simulink model "wscc9_transient_stability"  (R2024b)
settings: Solver=VariableStepAuto  StartTime=0.0  StopTime=2  MaxStep=1e-4  RelTol=1e-3
values from neighbouring files (symbols this model uses):
  E1 = E(1)    [wscc9_transient_init.m]
  E2 = E(2)    [wscc9_transient_init.m]
  E3 = E(3)    [wscc9_transient_init.m]
  f = 60    [wscc9_transient_init.m]
  H = [23.645 ; 6.4 ; 3.01]    [wscc9_transient_init.m]
  Pm1 = (Pg(1,1))    [wscc9_transient_init.m]
  Pm2 = (Pg(2,1))    [wscc9_transient_init.m]
  Pm3 = (Pg(3,1))    [wscc9_transient_init.m]
  Y2 = K-(L*inv(M)*LT)    [wscc9_transient_init.m]
  Y3 = K-(L*inv(M)*LT)    [wscc9_transient_init.m]
settings Model: Creator=Hussain  LastModifiedBy=Hussain
settings SolverCC: AlgebraicLoopSolver=TrustRegion
settings DataIOCC: ReturnWorkspaceOutputs=off
settings DebuggingCC: UnconnectedInputMsg=warning  UnconnectedOutputMsg=warning  UnconnectedLineMsg=warning  ArithmeticOperatorsInVariantConditions=warning
settings ModelReferenceCC: EnableRefExpFcnMdlSchedulingChecks=on
settings SFSimCC: SimUseLocalCustomCode=off  CustomCodeUndefinedFunction=UseInterfaceOnly
settings RTWCC: RTWUseLocalCustomCode=off  GPUComputeCapability=3.5
settings CodeAppCC: StateflowObjectComments=on

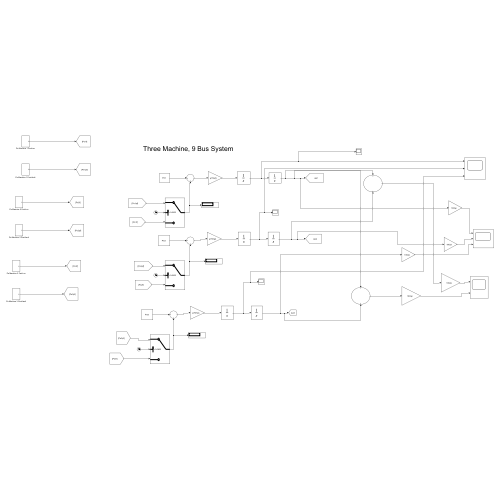
[thumbnail: Simulink's stored preview of the top-level diagram]
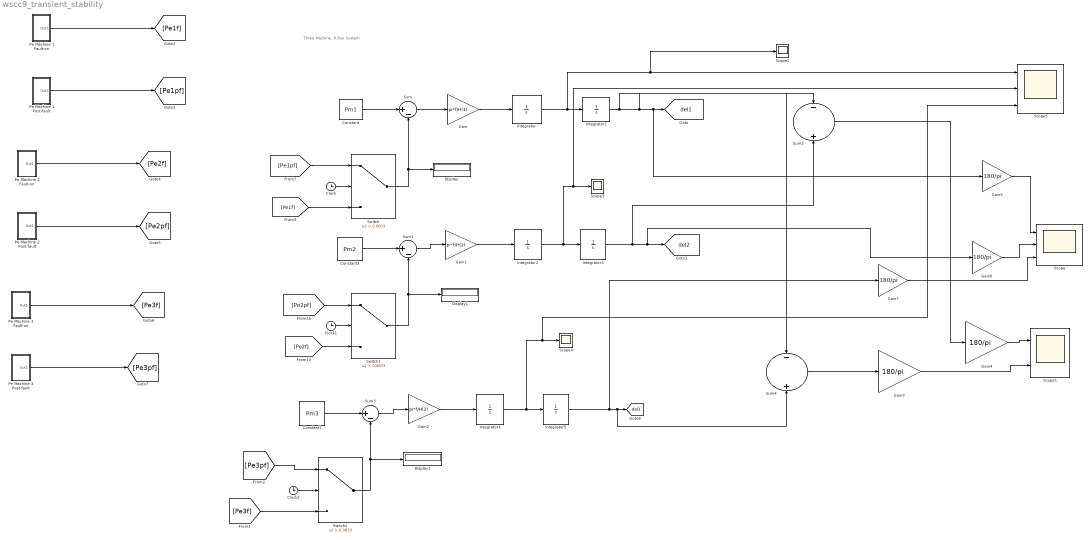
== system wscc9_transient_stability ==
  note: Three Machine, 9 Bus System
  Clock : Clock
  Clock1 : Clock
  Clock2 : Clock
  Constant : Constant  Value=Pm1
  Constant1 : Constant  Value=Pm3
  Constant3 : Constant  Value=Pm2
  Display : Display
  Display1 : Display
  Display2 : Display
  Gain : Gain  Gain=pi*f/H(1)
  Gain1 : Gain  Gain=pi*f/H(2)
  Gain2 : Gain  Gain=pi*f/H(3)
  Gain{3..7} (5 alike) : Gain  Gain=180/pi
  Integrator : Integrator
  Integrator1 : Integrator  InitialCondition=0.0396
  Integrator2 : Integrator
  Integrator3 : Integrator  InitialCondition=0.3447
  Integrator4 : Integrator
  Integrator5 : Integrator  InitialCondition=0.2301
  Pe Machine 1 Fault-on : Subsystem
  Pe Machine 1 Post-fault : Subsystem
  Pe Machine 2 Fault-on : Subsystem
  Pe Machine 2 Post-fault : Subsystem
  Pe Machine 3 Fault-on : Subsystem
  Pe Machine 3 Post-fault : Subsystem
  Scope : Scope  NumInputPorts=3
  Scope1 : Scope  NumInputPorts=2
  Scope2 : Scope
  Scope3 : Scope
  Scope4 : Scope
  Scope5 : Scope  NumInputPorts=3
  Sum : Sum  Inputs=|+-
  Sum1 : Sum  Inputs=|+-
  Sum2 : Sum  Inputs=-+
  Sum3 : Sum  Inputs=|+-
  Sum4 : Sum  Inputs=-+
  Switch : Switch  Criteria=u2 > Threshold  Threshold=0.0833  SaturateOnIntegerOverflow=off  InputSameDT=off
  Switch1 : Switch  Criteria=u2 > Threshold  Threshold=0.0833  SaturateOnIntegerOverflow=off  InputSameDT=off
  Switch2 : Switch  Criteria=u2 > Threshold  Threshold=0.0833  SaturateOnIntegerOverflow=off  InputSameDT=off
  tag scope: del1=global, del2=global, del3=global
  wires:
  Integrator/1 -> Scope5/1, Scope2/1, Integrator1/1
  Gain/1 -> Integrator/1
  Sum/1 -> Gain/1
  Constant/1 -> Sum/1
  Switch/1 -> Display/1, Sum/2
  Clock/1 -> Switch/2
  Integrator1/1 -> Sum4/1, Sum2/1, Gain5/1, [del1]
  Gain1/1 -> Integrator2/1
  Sum1/1 -> Gain1/1
  Constant3/1 -> Sum1/1
  Switch1/1 -> Display1/1, Sum1/2
  [Pe2pf] -> Switch1/1
  [Pe2f] -> Switch1/3
  Clock1/1 -> Switch1/2
  Integrator3/1 -> Sum2/2, Gain6/1, [del2]
  [Pe1f] -> Switch/3
  [Pe1pf] -> Switch/1
  Pe Machine 1 Fault-on/1(Out1) -> [Pe1f]
  Pe Machine 1 Post-fault/1(Out1) -> [Pe1pf]
  Integrator4/1 -> Scope5/3, Scope4/1, Integrator5/1
  Gain2/1 -> Integrator4/1
  Sum3/1 -> Gain2/1
  Constant1/1 -> Sum3/1
  Switch2/1 -> Sum3/2, Display2/1
  Clock2/1 -> Switch2/2
  Integrator5/1 -> Gain7/1, Sum4/2, [del3]
  Pe Machine 2 Fault-on/1(Out1) -> [Pe2f]
  Pe Machine 2 Post-fault/1(Out1) -> [Pe2pf]
  Pe Machine 3 Fault-on/1(Out1) -> [Pe3f]
  Pe Machine 3 Post-fault/1(Out1) -> [Pe3pf]
  [Pe3f] -> Switch2/3
  [Pe3pf] -> Switch2/1
  Sum2/1 -> Gain4/1
  Sum4/1 -> Gain3/1
  Integrator2/1 -> Scope5/2, Scope3/1, Integrator3/1
  Gain3/1 -> Scope1/2
  Gain4/1 -> Scope1/1
  Gain5/1 -> Scope/1
  Gain6/1 -> Scope/2
  Gain7/1 -> Scope/3

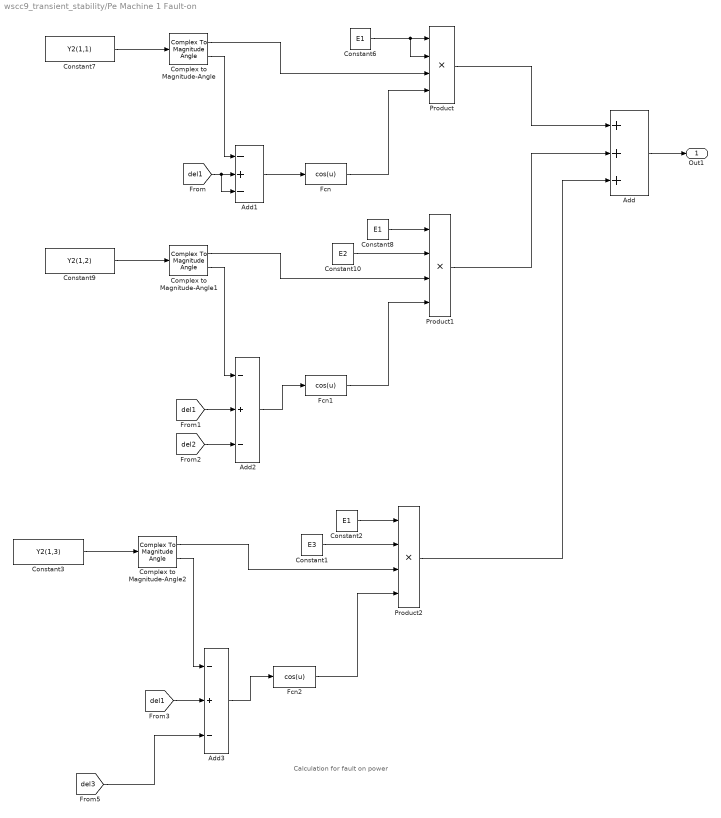
== system wscc9_transient_stability/Pe Machine 1 Fault-on ==
  note: Calculation for fault on power
  Add : Sum  Inputs=+++
  Add1 : Sum  Inputs=-+-
  Add2 : Sum  Inputs=-+-
  Add3 : Sum  Inputs=-+-
  Complex to Magnitude-Angle : ComplexToMagnitudeAngle
  Complex to Magnitude-Angle1 : ComplexToMagnitudeAngle
  Complex to Magnitude-Angle2 : ComplexToMagnitudeAngle
  Constant1 : Constant  Value=E3
  Constant10 : Constant  Value=E2
  Constant2 : Constant  Value=E1
  Constant3 : Constant  Value=Y2(1,3)
  Constant6 : Constant  Value=E1
  Constant7 : Constant  Value=Y2(1,1)
  Constant8 : Constant  Value=E1
  Constant9 : Constant  Value=Y2(1,2)
  Fcn : Fcn  Expr=cos(u)
  Fcn1 : Fcn  Expr=cos(u)
  Fcn2 : Fcn  Expr=cos(u)
  Product : Product  Inputs=4
  Product1 : Product  Inputs=4
  Product2 : Product  Inputs=4
  Out1 : Outport
  wires:
  Constant7/1 -> Complex to Magnitude-Angle/1
  Fcn/1 -> Product/4
  Complex to Magnitude-Angle1/1 -> Product1/3
  [del1] -> Add2/2
  Add2/1 -> Fcn1/1
  Complex to Magnitude-Angle1/2 -> Add2/1
  Fcn1/1 -> Product1/4
  Constant8/1 -> Product1/1
  Constant9/1 -> Complex to Magnitude-Angle1/1
  Product1/1 -> Add/2
  Constant6/1 -> Product/2, Product/1
  Add1/1 -> Fcn/1
  Complex to Magnitude-Angle/1 -> Product/3
  Add/1 -> Out1/1
  Product/1 -> Add/1
  [del2] -> Add2/3
  Constant10/1 -> Product1/2
  Complex to Magnitude-Angle/2 -> Add1/1
  [del1] -> Add1/3, Add1/2
  Complex to Magnitude-Angle2/1 -> Product2/3
  [del1] -> Add3/2
  Add3/1 -> Fcn2/1
  Complex to Magnitude-Angle2/2 -> Add3/1
  Fcn2/1 -> Product2/4
  Constant2/1 -> Product2/1
  Constant3/1 -> Complex to Magnitude-Angle2/1
  [del3] -> Add3/3
  Constant1/1 -> Product2/2
  Product2/1 -> Add/3

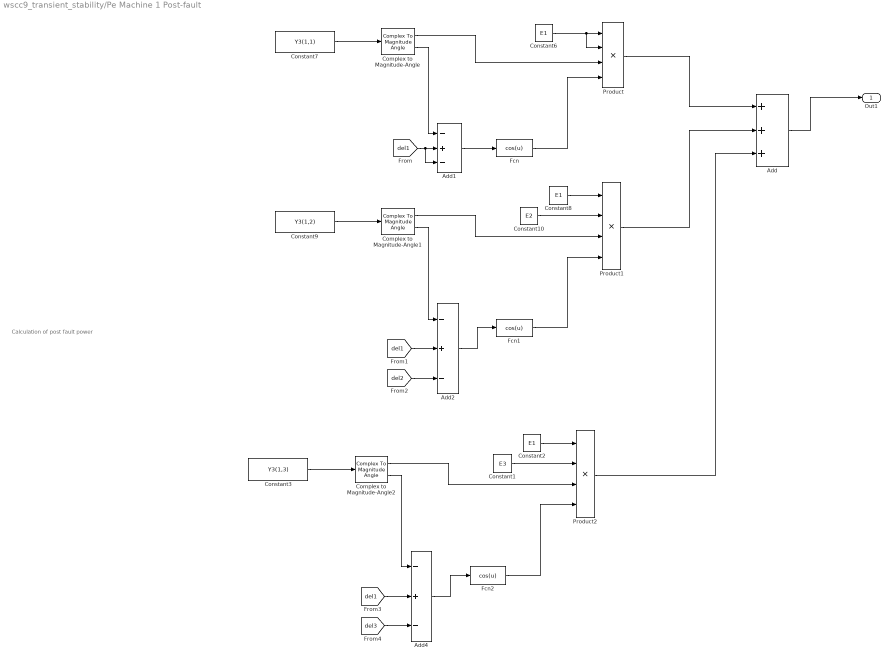
== system wscc9_transient_stability/Pe Machine 1 Post-fault ==
  note: Calculation of post fault power
  Add : Sum  Inputs=+++
  Add1 : Sum  Inputs=-+-
  Add2 : Sum  Inputs=-+-
  Add4 : Sum  Inputs=-+-
  Complex to Magnitude-Angle : ComplexToMagnitudeAngle
  Complex to Magnitude-Angle1 : ComplexToMagnitudeAngle
  Complex to Magnitude-Angle2 : ComplexToMagnitudeAngle
  Constant1 : Constant  Value=E3
  Constant10 : Constant  Value=E2
  Constant2 : Constant  Value=E1
  Constant3 : Constant  Value=Y3(1,3)
  Constant6 : Constant  Value=E1
  Constant7 : Constant  Value=Y3(1,1)
  Constant8 : Constant  Value=E1
  Constant9 : Constant  Value=Y3(1,2)
  Fcn : Fcn  Expr=cos(u)
  Fcn1 : Fcn  Expr=cos(u)
  Fcn2 : Fcn  Expr=cos(u)
  Product : Product  Inputs=4
  Product1 : Product  Inputs=4
  Product2 : Product  Inputs=4
  Out1 : Outport
  wires:
  Constant7/1 -> Complex to Magnitude-Angle/1
  Fcn/1 -> Product/4
  Complex to Magnitude-Angle1/1 -> Product1/3
  [del1] -> Add2/2
  Add2/1 -> Fcn1/1
  Complex to Magnitude-Angle1/2 -> Add2/1
  Fcn1/1 -> Product1/4
  Constant8/1 -> Product1/1
  Constant9/1 -> Complex to Magnitude-Angle1/1
  Product1/1 -> Add/2
  Constant6/1 -> Product/2, Product/1
  Add1/1 -> Fcn/1
  Complex to Magnitude-Angle/1 -> Product/3
  Add/1 -> Out1/1
  Product/1 -> Add/1
  [del2] -> Add2/3
  Constant10/1 -> Product1/2
  Complex to Magnitude-Angle/2 -> Add1/1
  [del1] -> Add1/3, Add1/2
  Complex to Magnitude-Angle2/1 -> Product2/3
  [del1] -> Add4/2
  Add4/1 -> Fcn2/1
  Complex to Magnitude-Angle2/2 -> Add4/1
  Fcn2/1 -> Product2/4
  Constant2/1 -> Product2/1
  Constant3/1 -> Complex to Magnitude-Angle2/1
  [del3] -> Add4/3
  Constant1/1 -> Product2/2
  Product2/1 -> Add/3

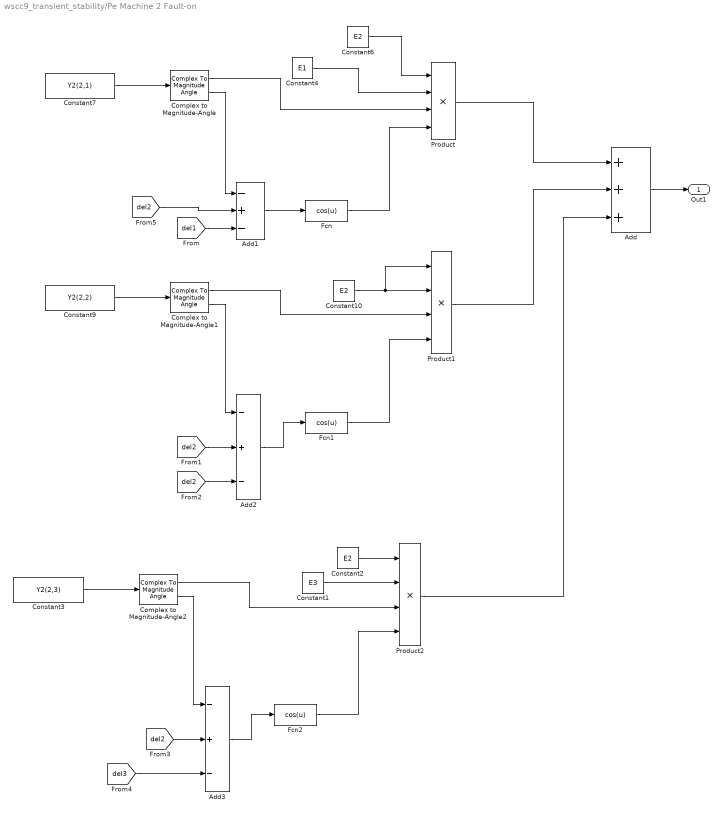
== system wscc9_transient_stability/Pe Machine 2 Fault-on ==
  Add : Sum  Inputs=+++
  Add1 : Sum  Inputs=-+-
  Add2 : Sum  Inputs=-+-
  Add3 : Sum  Inputs=-+-
  Complex to Magnitude-Angle : ComplexToMagnitudeAngle
  Complex to Magnitude-Angle1 : ComplexToMagnitudeAngle
  Complex to Magnitude-Angle2 : ComplexToMagnitudeAngle
  Constant1 : Constant  Value=E3
  Constant10 : Constant  Value=E2
  Constant2 : Constant  Value=E2
  Constant3 : Constant  Value=Y2(2,3)
  Constant4 : Constant  Value=E1
  Constant6 : Constant  Value=E2
  Constant7 : Constant  Value=Y2(2,1)
  Constant9 : Constant  Value=Y2(2,2)
  Fcn : Fcn  Expr=cos(u)
  Fcn1 : Fcn  Expr=cos(u)
  Fcn2 : Fcn  Expr=cos(u)
  Product : Product  Inputs=4
  Product1 : Product  Inputs=4
  Product2 : Product  Inputs=4
  Out1 : Outport
  wires:
  Constant7/1 -> Complex to Magnitude-Angle/1
  Fcn/1 -> Product/4
  Complex to Magnitude-Angle1/1 -> Product1/3
  [del2] -> Add2/2
  Add2/1 -> Fcn1/1
  Complex to Magnitude-Angle1/2 -> Add2/1
  Fcn1/1 -> Product1/4
  Constant10/1 -> Product1/1, Product1/2
  Constant9/1 -> Complex to Magnitude-Angle1/1
  Product1/1 -> Add/2
  Constant6/1 -> Product/1
  Add1/1 -> Fcn/1
  Complex to Magnitude-Angle/1 -> Product/3
  Add/1 -> Out1/1
  Product/1 -> Add/1
  [del2] -> Add2/3
  Complex to Magnitude-Angle/2 -> Add1/1
  Complex to Magnitude-Angle2/1 -> Product2/3
  [del2] -> Add3/2
  Add3/1 -> Fcn2/1
  Complex to Magnitude-Angle2/2 -> Add3/1
  Fcn2/1 -> Product2/4
  Constant2/1 -> Product2/1
  Constant3/1 -> Complex to Magnitude-Angle2/1
  [del3] -> Add3/3
  Constant1/1 -> Product2/2
  Product2/1 -> Add/3
  Constant4/1 -> Product/2
  [del1] -> Add1/3
  [del2] -> Add1/2

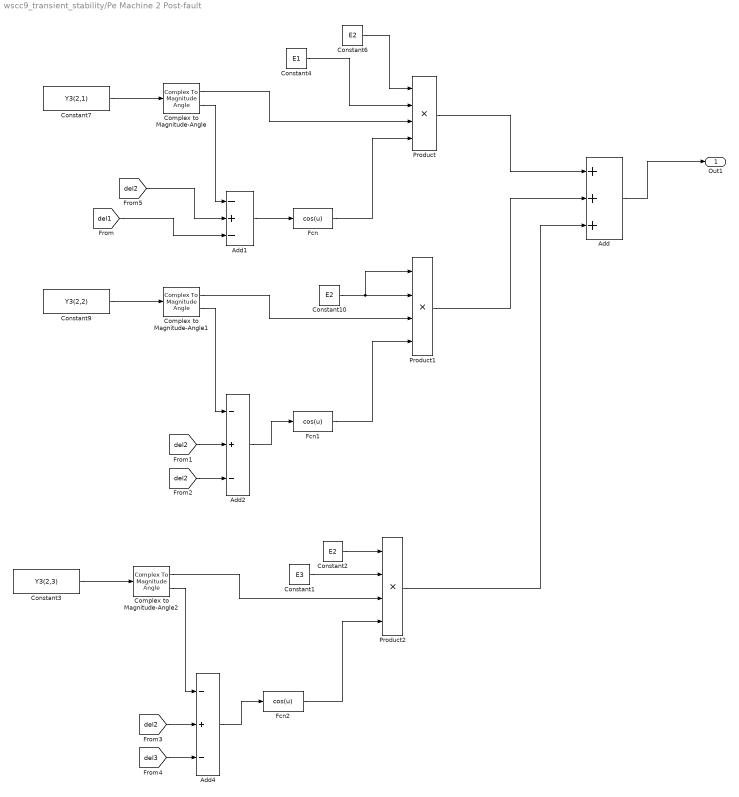
== system wscc9_transient_stability/Pe Machine 2 Post-fault ==
  Add : Sum  Inputs=+++
  Add1 : Sum  Inputs=-+-
  Add2 : Sum  Inputs=-+-
  Add4 : Sum  Inputs=-+-
  Complex to Magnitude-Angle : ComplexToMagnitudeAngle
  Complex to Magnitude-Angle1 : ComplexToMagnitudeAngle
  Complex to Magnitude-Angle2 : ComplexToMagnitudeAngle
  Constant1 : Constant  Value=E3
  Constant10 : Constant  Value=E2
  Constant2 : Constant  Value=E2
  Constant3 : Constant  Value=Y3(2,3)
  Constant4 : Constant  Value=E1
  Constant6 : Constant  Value=E2
  Constant7 : Constant  Value=Y3(2,1)
  Constant9 : Constant  Value=Y3(2,2)
  Fcn : Fcn  Expr=cos(u)
  Fcn1 : Fcn  Expr=cos(u)
  Fcn2 : Fcn  Expr=cos(u)
  Product : Product  Inputs=4
  Product1 : Product  Inputs=4
  Product2 : Product  Inputs=4
  Out1 : Outport
  wires:
  Constant7/1 -> Complex to Magnitude-Angle/1
  Fcn/1 -> Product/4
  Complex to Magnitude-Angle1/1 -> Product1/3
  [del2] -> Add2/2
  Add2/1 -> Fcn1/1
  Complex to Magnitude-Angle1/2 -> Add2/1
  Fcn1/1 -> Product1/4
  Constant10/1 -> Product1/1, Product1/2
  Constant9/1 -> Complex to Magnitude-Angle1/1
  Product1/1 -> Add/2
  Constant6/1 -> Product/1
  Add1/1 -> Fcn/1
  Complex to Magnitude-Angle/1 -> Product/3
  Add/1 -> Out1/1
  Product/1 -> Add/1
  [del2] -> Add2/3
  Complex to Magnitude-Angle/2 -> Add1/1
  Complex to Magnitude-Angle2/1 -> Product2/3
  [del2] -> Add4/2
  Add4/1 -> Fcn2/1
  Complex to Magnitude-Angle2/2 -> Add4/1
  Fcn2/1 -> Product2/4
  Constant2/1 -> Product2/1
  Constant3/1 -> Complex to Magnitude-Angle2/1
  [del3] -> Add4/3
  Constant1/1 -> Product2/2
  Product2/1 -> Add/3
  Constant4/1 -> Product/2
  [del1] -> Add1/3
  [del2] -> Add1/2

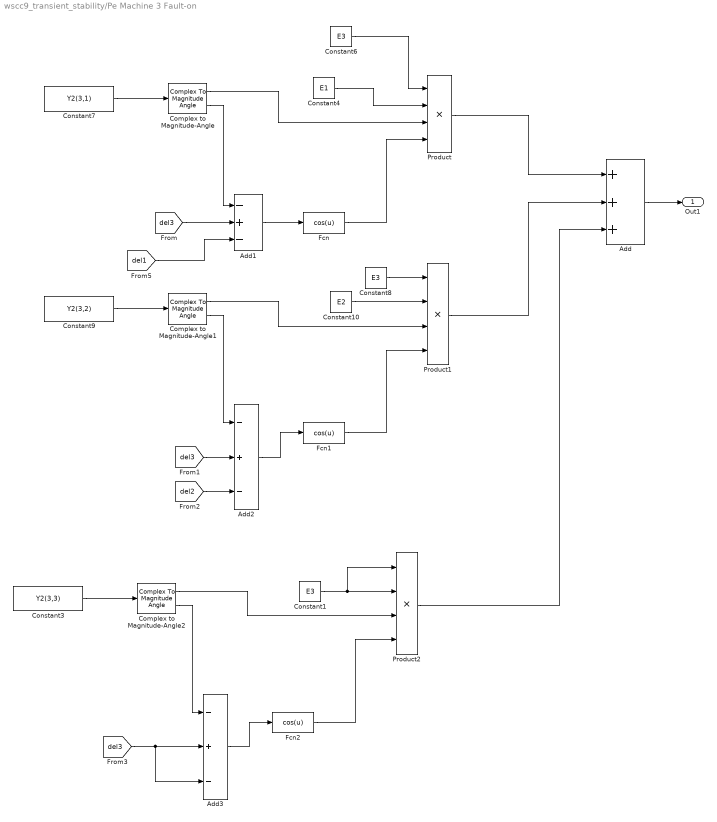
== system wscc9_transient_stability/Pe Machine 3 Fault-on ==
  Add : Sum  Inputs=+++
  Add1 : Sum  Inputs=-+-
  Add2 : Sum  Inputs=-+-
  Add3 : Sum  Inputs=-+-
  Complex to Magnitude-Angle : ComplexToMagnitudeAngle
  Complex to Magnitude-Angle1 : ComplexToMagnitudeAngle
  Complex to Magnitude-Angle2 : ComplexToMagnitudeAngle
  Constant1 : Constant  Value=E3
  Constant10 : Constant  Value=E2
  Constant3 : Constant  Value=Y2(3,3)
  Constant4 : Constant  Value=E1
  Constant6 : Constant  Value=E3
  Constant7 : Constant  Value=Y2(3,1)
  Constant8 : Constant  Value=E3
  Constant9 : Constant  Value=Y2(3,2)
  Fcn : Fcn  Expr=cos(u)
  Fcn1 : Fcn  Expr=cos(u)
  Fcn2 : Fcn  Expr=cos(u)
  Product : Product  Inputs=4
  Product1 : Product  Inputs=4
  Product2 : Product  Inputs=4
  Out1 : Outport
  wires:
  Constant7/1 -> Complex to Magnitude-Angle/1
  Fcn/1 -> Product/4
  Complex to Magnitude-Angle1/1 -> Product1/3
  [del3] -> Add2/2
  Add2/1 -> Fcn1/1
  Complex to Magnitude-Angle1/2 -> Add2/1
  Fcn1/1 -> Product1/4
  Constant8/1 -> Product1/1
  Constant9/1 -> Complex to Magnitude-Angle1/1
  Product1/1 -> Add/2
  Constant6/1 -> Product/1
  Add1/1 -> Fcn/1
  Complex to Magnitude-Angle/1 -> Product/3
  Add/1 -> Out1/1
  Product/1 -> Add/1
  [del2] -> Add2/3
  Constant10/1 -> Product1/2
  Complex to Magnitude-Angle/2 -> Add1/1
  [del3] -> Add1/2
  Complex to Magnitude-Angle2/1 -> Product2/3
  Add3/1 -> Fcn2/1
  Complex to Magnitude-Angle2/2 -> Add3/1
  Fcn2/1 -> Product2/4
  Constant1/1 -> Product2/1, Product2/2
  Constant3/1 -> Complex to Magnitude-Angle2/1
  [del3] -> Add3/3, Add3/2
  Product2/1 -> Add/3
  Constant4/1 -> Product/2
  [del1] -> Add1/3

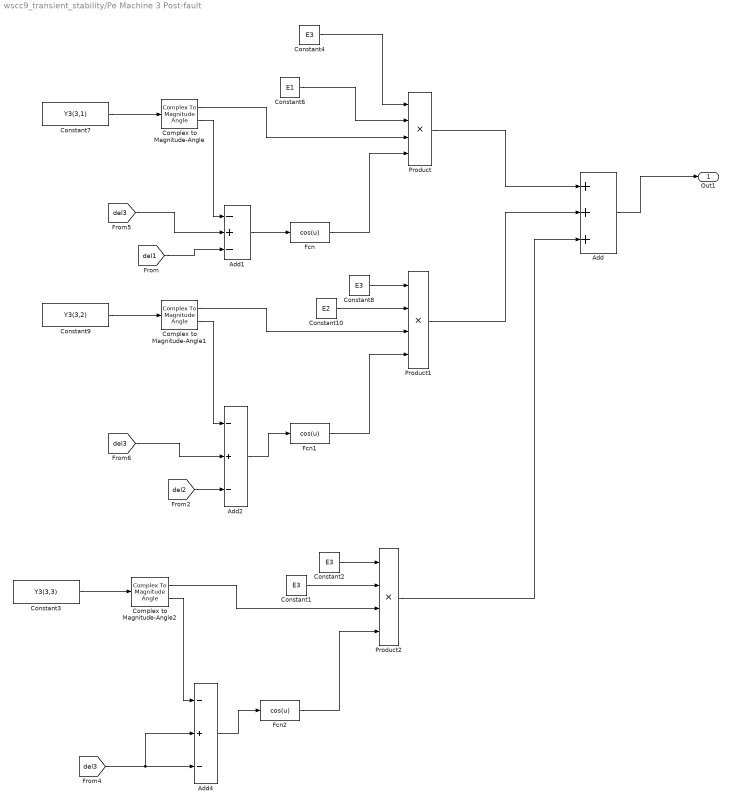
== system wscc9_transient_stability/Pe Machine 3 Post-fault ==
  Add : Sum  Inputs=+++
  Add1 : Sum  Inputs=-+-
  Add2 : Sum  Inputs=-+-
  Add4 : Sum  Inputs=-+-
  Complex to Magnitude-Angle : ComplexToMagnitudeAngle
  Complex to Magnitude-Angle1 : ComplexToMagnitudeAngle
  Complex to Magnitude-Angle2 : ComplexToMagnitudeAngle
  Constant{1..2,4,8} (4 alike) : Constant  Value=E3
  Constant10 : Constant  Value=E2
  Constant3 : Constant  Value=Y3(3,3)
  Constant6 : Constant  Value=E1
  Constant7 : Constant  Value=Y3(3,1)
  Constant9 : Constant  Value=Y3(3,2)
  Fcn : Fcn  Expr=cos(u)
  Fcn1 : Fcn  Expr=cos(u)
  Fcn2 : Fcn  Expr=cos(u)
  Product : Product  Inputs=4
  Product1 : Product  Inputs=4
  Product2 : Product  Inputs=4
  Out1 : Outport
  wires:
  Constant7/1 -> Complex to Magnitude-Angle/1
  Fcn/1 -> Product/4
  Complex to Magnitude-Angle1/1 -> Product1/3
  [del3] -> Add2/2
  Add2/1 -> Fcn1/1
  Complex to Magnitude-Angle1/2 -> Add2/1
  Fcn1/1 -> Product1/4
  Constant8/1 -> Product1/1
  Constant9/1 -> Complex to Magnitude-Angle1/1
  Product1/1 -> Add/2
  Add1/1 -> Fcn/1
  Complex to Magnitude-Angle/1 -> Product/3
  Add/1 -> Out1/1
  Product/1 -> Add/1
  [del2] -> Add2/3
  Constant10/1 -> Product1/2
  Complex to Magnitude-Angle/2 -> Add1/1
  [del1] -> Add1/3
  Complex to Magnitude-Angle2/1 -> Product2/3
  [del3] -> Add4/2, Add4/3
  Add4/1 -> Fcn2/1
  Complex to Magnitude-Angle2/2 -> Add4/1
  Fcn2/1 -> Product2/4
  Constant2/1 -> Product2/1
  Constant3/1 -> Complex to Magnitude-Angle2/1
  Constant1/1 -> Product2/2
  Product2/1 -> Add/3
  Constant6/1 -> Product/2
  Constant4/1 -> Product/1
  [del3] -> Add1/2
